simulink model "Physics_Testbench"  (R2025b)
settings: Solver=ode4  StartTime=0.0  StopTime=0.5  FixedStep=plantTs  RelTol=1e-3
undefined symbols (not defined in the file): tauGravity
settings Model: Creator=Compu  LastModifiedBy=Compu

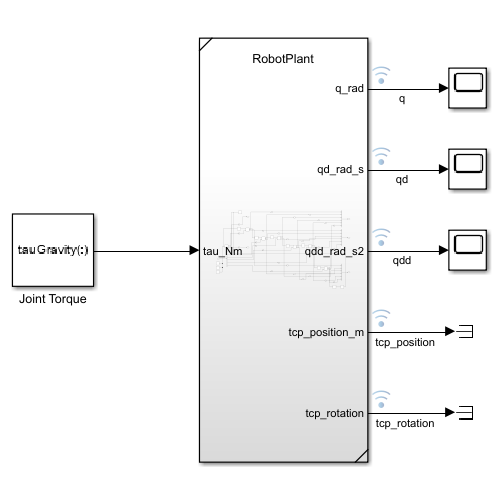
[thumbnail: Simulink's stored preview of the top-level diagram]
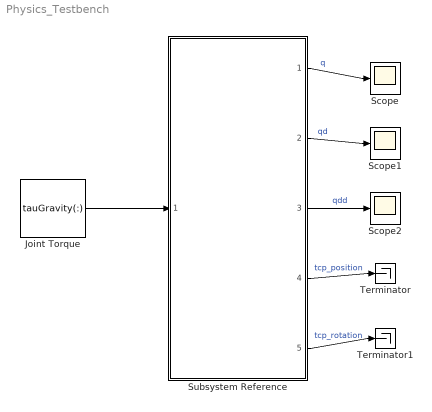
== system Physics_Testbench ==
  Joint Torque : Constant  Value=tauGravity(:)
  Scope : Scope
  Scope1 : Scope
  Scope2 : Scope
      settings: DataLoggingVariableName=ScopeData2
  Subsystem Reference : Subsystem  ReferencedSubsystem=RobotPlant
  Terminator : Terminator
  Terminator1 : Terminator
  wires:
  Subsystem Reference/1 -> Scope/1  "q"
  Subsystem Reference/2 -> Scope1/1  "qd"
  Subsystem Reference/3 -> Scope2/1  "qdd"
  Subsystem Reference/4 -> Terminator/1  "tcp_position"
  Subsystem Reference/5 -> Terminator1/1  "tcp_rotation"
  Joint Torque/1 -> Subsystem Reference/1
